simulink model "weighted_adder"  (R2026b)
settings: Solver=FixedStepDiscrete  FixedStep=0.1
undefined symbols (not defined in the file): feedback_gain
settings Model: Creator=Fasih  LastModifiedBy=Fasih

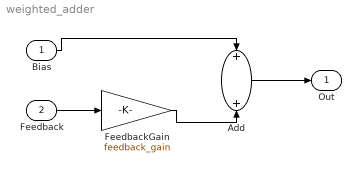
== system weighted_adder ==
  Bias : Inport
  Feedback : Inport  Port=2
  Add : Sum
  FeedbackGain : Gain  Gain=feedback_gain
  Out : Outport
  wires:
  Bias/1 -> Add/1
  Feedback/1 -> FeedbackGain/1
  FeedbackGain/1 -> Add/2
  Add/1 -> Out/1
